simulink model "landing"  (R2026b)
settings: Solver=VariableStepAuto  StopTime=120.0
undefined symbols (not defined in the file): p
settings Model: Creator=lorenzomonti  LastModifiedBy=lorenzomonti

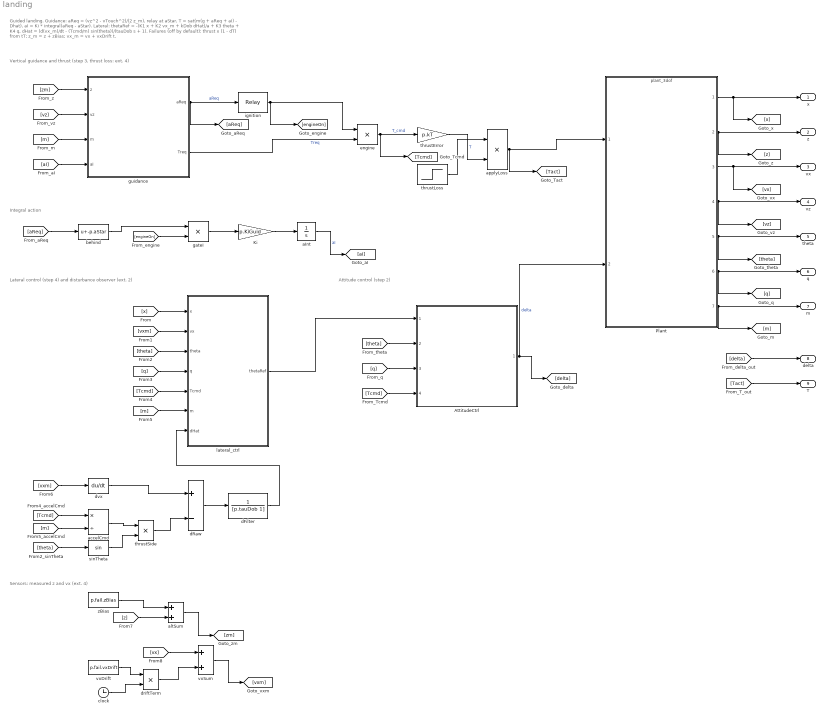
== system landing ==
  note: Vertical guidance and thrust (step 3, thrust loss: ext. 4)
  note: Integral action
  note: Lateral control (step 4) and disturbance observer (ext. 2)
  note: Attitude control (step 2)
  note: Sensors: measured z and vx (ext. 4)
  note: Guided landing. Guidance: aReq = (vz^2 - vTouch^2)/(2 z_m), relay at aStar, T = sat(m(g + aReq + aI) - Dhat), aI = Ki * integral(aReq - aStar).
      | Lateral: thetaRef = -(K1 x + K2 vx_m + kDob dHat)/a + K3 theta + K4 q, dHat = (d(vx_m)/dt - (Tcmd/m) sin(theta))/(tauDob s + 1).
      | Failures (off by default): thrust x (1 - dT) from tT; z_m = z + zBias; vx_m = vx + vxDrift t.
  AttitudeCtrl : Subsystem  ReferencedSubsystem=attitude_ctrl
  Ki : Gain  Gain=p.KiGuid
  Plant : ModelReference  ModelNameDialog=plant_3dof  SimulationMode=Normal  ModelReferenceVersion=1.17
  aInt : Integrator
  accelCmd : Product  Inputs=*/
  altSum : Sum
  applyLoss : Product
  behind : Bias  Bias=-p.aStar  SaturateOnIntegerOverflow=off
  clock : Clock
  dFilter : TransferFcn  Denominator=[p.tauDob 1]
  dRaw : Sum  Inputs=+-
  driftTerm : Product
  dvx : Derivative
  engine : Product
  gateI : Product
  guidance : MATLAB Function  TreatAsAtomicUnit=on
  ignition : Relay  OnSwitchValue=p.aStar  OffSwitchValue=p.aOff
  lateral_ctrl : MATLAB Function  TreatAsAtomicUnit=on
  sinTheta : Trigonometry
  thrustError : Gain  Gain=p.kT
  thrustLoss : Step  Time=p.fail.tT  InitialValue=1  FinalValue=1 - p.fail.dT  SampleTime=0
  thrustSide : Product
  vxDrift : Constant  Value=p.fail.vxDrift
  vxSum : Sum
  zBias : Constant  Value=p.fail.zBias
  x : Outport
  z : Outport  Port=2
  vx : Outport  Port=3
  vz : Outport  Port=4
  theta : Outport  Port=5
  q : Outport  Port=6
  m : Outport  Port=7
  delta : Outport  Port=8
  T : Outport  Port=9
  wires:
  vxSum/1 -> [vxm]
  driftTerm/1 -> vxSum/2
  [vx] -> vxSum/1
  altSum/1 -> [zm]
  [z] -> altSum/2
  zBias/1 -> altSum/1
  clock/1 -> driftTerm/2
  vxDrift/1 -> driftTerm/1
  applyLoss/1 -> Plant/1, [Tact]
  thrustError/1 -> applyLoss/2  "T"
  thrustLoss/1 -> applyLoss/1
  lateral_ctrl/1(thetaRef) -> AttitudeCtrl/1
  [Tcmd] -> AttitudeCtrl/4
  [aI] -> guidance/4(aI)
  guidance/1(aReq) -> ignition/1, [aReq]  "aReq"
  Plant/4 -> vz/1, [vz]
  AttitudeCtrl/1 -> [delta], Plant/2  "delta"
  [theta] -> lateral_ctrl/3(theta)
  [theta] -> sinTheta/1
  Plant/1 -> [x], x/1
  guidance/2(Treq) -> engine/2  "Treq"
  [Tcmd] -> lateral_ctrl/5(Tcmd)
  [Tcmd] -> accelCmd/1
  [theta] -> AttitudeCtrl/2
  dRaw/1 -> dFilter/1
  engine/1 -> thrustError/1, [Tcmd]  "T_cmd"
  [q] -> AttitudeCtrl/3
  [zm] -> guidance/1(z)
  ignition/1 -> engine/1, [engineOn]
  gateI/1 -> Ki/1
  dFilter/1 -> lateral_ctrl/7(dHat)
  [aReq] -> behind/1
  Ki/1 -> aInt/1
  [Tact] -> T/1
  [m] -> guidance/3(m)
  thrustSide/1 -> dRaw/2
  [vxm] -> lateral_ctrl/2(vx)
  behind/1 -> gateI/1
  [engineOn] -> gateI/2
  [vxm] -> dvx/1
  aInt/1 -> [aI]  "aI"
  Plant/7 -> m/1, [m]
  [delta] -> delta/1
  [vz] -> guidance/2(vz)
  [m] -> lateral_ctrl/6(m)
  [m] -> accelCmd/2
  accelCmd/1 -> thrustSide/1
  sinTheta/1 -> thrustSide/2
  dvx/1 -> dRaw/1
  Plant/3 -> [vx], vx/1
  [x] -> lateral_ctrl/1(x)
  [q] -> lateral_ctrl/4(q)
  Plant/5 -> theta/1, [theta]
  Plant/2 -> z/1, [z]
  Plant/6 -> q/1, [q]

== matlab function landing/lateral_ctrl ==
  data: x input; thetaRef output; vx input; theta input; q input; Tcmd input; m input; dHat input; p parameter
function thetaRef = lateral_ctrl(x, vx, theta, q, Tcmd, m,  dHat, p)

if Tcmd <= 0
    thetaRef = 0;
    return
end

a = (Tcmd)/m;

thetaRef = -(p.Klat(1)*x + p.Klat(2)*vx)/a ...
           + p.Klat(3)*theta + p.Klat(4)*q ...
           - p.kDob*dHat/a;

thetaRef = min(max(thetaRef, -p.thetaRefMax), p.thetaRefMax);

== matlab function landing/guidance ==
  data: z input; aReq output; Treq output; vz input; m input; aI input; p parameter
function [aReq, Treq] = guidance(z, vz, m, aI, p)

if z > p.zGate 
    aReq = (vz^2 - p.vGate^2)/(2 * max((z - p.zGate), p.zMin));
else
    aReq = (vz^2 - p.vTouch^2)/(2 * max(z, p.zMin));
end

Dhat = 0.5 * p.rho0 * exp(-z/p.H) * p.CDhat * p.A * vz^2;

if z > p.zGate
    Treq = min(max(m * (p.g + aReq + aI) - Dhat, p.Tmin), p.Tmax);
else
    Treq = min(max(m * (p.g + aReq) - Dhat, p.Tmin), p.Tmax);
end
